simulink model "s_c_nbe_m32k"  (R2018a)
settings: Solver=VariableStepDiscrete  StartTime=0.0  StopTime=1000  RelTol=1e-3
undefined symbols (not defined in the file): fft_stages, n_taps, output_bits, pfb_coeff_gen_calc, xengbits
libraries: xbsIndex_r4 x23714, casper_library_misc x17, xps_library x4, casper_library_scopes x4, xbsReplacements_r4 x4
(part 8 of 171)

== system s_c_nbe_m32k/cd_hmc ==
  note: new delay values/enables come aligned
      | with data, need to be one cycle before
      | so new delay value gets loaded at the
      | same time as data, so delay data path
      | by one cycle
  sync_in : Inport
  din : Inport  Port=2
  en : Inport  Port=3
  delay_val : Inport  Port=4
  load_val : Inport  Port=5
  sync_in1 : Inport  Port=6
  din1 : Inport  Port=7
  en1 : Inport  Port=8
  delay_val1 : Inport  Port=9
  load_val1 : Inport  Port=10
  Constant : xbsIndex_r4/Constant  const=2^(n_bits_fft-3-1)  gui_display_data_type=Fixed-point  arith_type=Unsigned  n_bits=n_bits_fft-3  bin_pt=0  preci_type=Single  exp_width=8  frac_width=24  explicit_period=on  period=1  equ=P=C  opselect=C  inp2=PCIN>>17  opr=+  inp1=P  carry=CIN  dbl_ovrd=off  block_type=constant
  Constant1 : xbsIndex_r4/Constant  const=2^(n_bits_fft-3-1)  gui_display_data_type=Fixed-point  arith_type=Unsigned  n_bits=n_bits_fft-3  bin_pt=0  preci_type=Single  exp_width=8  frac_width=24  explicit_period=on  period=1  equ=P=C  opselect=C  inp2=PCIN>>17  opr=+  inp1=P  carry=CIN  dbl_ovrd=off  block_type=constant
  Constant2 : xbsIndex_r4/Constant  const=0  gui_display_data_type=Boolean  arith_type=Boolean  n_bits=1  bin_pt=0  preci_type=Single  exp_width=8  frac_width=24  explicit_period=on  period=1  equ=P=C  opselect=C  inp2=PCIN>>17  opr=+  inp1=P  carry=CIN  dbl_ovrd=off  block_type=constant
      settings: block_version=11.4
  Constant53 : xbsIndex_r4/Constant  const=0  gui_display_data_type=Boolean  arith_type=Boolean  n_bits=1  bin_pt=0  preci_type=Single  exp_width=8  frac_width=24  explicit_period=on  period=1  equ=P=C  opselect=C  inp2=PCIN>>17  opr=+  inp1=P  carry=CIN  dbl_ovrd=off  block_type=constant
      settings: block_version=11.4
  Delay : xbsIndex_r4/Delay  rst=off  infoeditControl=Selection of Reset will increase slice count due to use of real FFs and instead of SRLs  en=on  latency=1  reg_retiming=off  dbl_ovrd=off  block_type=delay
  Delay{1..4,6..19,21..34,36..39} (36 alike) : xbsIndex_r4/Delay  rst=off  infoeditControl=Selection of Reset will increase slice count due to use of real FFs and instead of SRLs  en=off  latency=1  reg_retiming=on  dbl_ovrd=off  block_type=delay
  Delay20 : xbsIndex_r4/Delay  rst=off  infoeditControl=Selection of Reset will increase slice count due to use of real FFs and instead of SRLs  en=on  latency=1  reg_retiming=off  dbl_ovrd=off  block_type=delay
  Delay35 : xbsIndex_r4/Delay  rst=off  infoeditControl=Selection of Reset will increase slice count due to use of real FFs and instead of SRLs  en=off  latency=1  reg_retiming=off  dbl_ovrd=off  block_type=delay
  Delay5 : xbsIndex_r4/Delay  rst=off  infoeditControl=Selection of Reset will increase slice count due to use of real FFs and instead of SRLs  en=off  latency=1  reg_retiming=off  dbl_ovrd=off  block_type=delay
  Logical : xbsIndex_r4/Logical  logical_function=AND  inputs=2  en=off  latency=1  precision=Full  arith_type=Unsigned  n_bits=16  bin_pt=0  align_bp=on  dbl_ovrd=off  block_type=logical
  Logical1 : xbsIndex_r4/Logical  logical_function=AND  inputs=2  en=off  latency=1  precision=Full  arith_type=Unsigned  n_bits=16  bin_pt=0  align_bp=on  dbl_ovrd=off  block_type=logical
  Slice1 : xbsIndex_r4/Slice  nbits=4  boolean_output=off  mode=Two Bit Locations  bit1=0  base1=MSB of Input  bit0=4  base0=LSB of Input  dbl_ovrd=off  block_type=slice
  Slice2 : xbsIndex_r4/Slice  nbits=4  boolean_output=off  mode=Two Bit Locations  bit1=0  base1=MSB of Input  bit0=4  base0=LSB of Input  dbl_ovrd=off  block_type=slice
  bus_expand1 : Subsystem  mask(bus_expand){mode=divisions of arbitrary size, outputNum=1, outputWidth=[64 64 16 16], outputBinaryPt=[32 32 15 15], outputArithmeticType=[1 1 1 1], show_format=off, outputToWorkspace=off, variablePrefix=out, outputToModelAsWell=on}
      mask prompts: outputNum "Number of outputs:"; outputWidth "Output width [msb ... lsb]:"; outputBinaryPt "Output binary point position [msb ... lsb]:"; outputArithmeticType "Output arithmetic type (ufix=0, fix=1, bool=2) [msb ... lsb]:"; show_format "Print format string?"; outputToWorkspace "Output to workspace?"; variablePrefix "Variable name prefix:"; outputToModelAsWell "Output to model as well?"
      mask help:
      | Expands a 'bus' made using a bus_create or Xilinx
      | concat block.
      | The input will be divided into the specified number
      | of outputs with the specified arithmetic types.
      | Divisions are made from most significant bit.
      mask init: same as s_c_nbe_m32k/bus_expand1
      settings: AttributesFormatString=4 outputs
      mask TypeOptions mode: divisions of equal size | divisions of arbitrary size
      mask Callback mode: bus_expand_callback();
      mask Callback outputWidth: bus_expand_callback();
      mask Callback outputToWorkspace: bus_expand_callback();
  bus_expand2 : Subsystem  mask(bus_expand){mode=divisions of arbitrary size, outputNum=1, outputWidth=[64 64 16 16], outputBinaryPt=[32 32 15 15], outputArithmeticType=[1 1 1 1], show_format=off, outputToWorkspace=off, variablePrefix=out, outputToModelAsWell=on}
      mask prompts: outputNum "Number of outputs:"; outputWidth "Output width [msb ... lsb]:"; outputBinaryPt "Output binary point position [msb ... lsb]:"; outputArithmeticType "Output arithmetic type (ufix=0, fix=1, bool=2) [msb ... lsb]:"; show_format "Print format string?"; outputToWorkspace "Output to workspace?"; variablePrefix "Variable name prefix:"; outputToModelAsWell "Output to model as well?"
      mask help:
      | Expands a 'bus' made using a bus_create or Xilinx
      | concat block.
      | The input will be divided into the specified number
      | of outputs with the specified arithmetic types.
      | Divisions are made from most significant bit.
      mask init: same as s_c_nbe_m32k/bus_expand1
      settings: AttributesFormatString=4 outputs
      mask TypeOptions mode: divisions of equal size | divisions of arbitrary size
      mask Callback mode: bus_expand_callback();
      mask Callback outputWidth: bus_expand_callback();
      mask Callback outputToWorkspace: bus_expand_callback();
  delay_gen0 : Subsystem  mask{fft_len=n_bits_fft-1, add_latency=1, data_bits=10 * 8, n_bits_index=n_bits_fft-3, lookup_bits=11, cd_bits=n_bits_cd, delay_bits=n_bits_cd+32, delay_bin_pt=32, max_delay_rate=23, min_delay_rate=38, phase_bits=16, max_phase_rate=23, min_phase_rate=38}
      mask prompts: fft_len "Effective FFT size (2^?)"; add_latency "Add latency"; data_bits "Data width"; n_bits_index "Index width"; lookup_bits "DDS lookup table resolution (2*pi/2^?)"; cd_bits "Coarse delay range (2^? bits)"; delay_bits "Input delay resolution (bits)"; delay_bin_pt "Input delay binary point"; max_delay_rate "Max delay update rate (1/2^? samples/sample)"; min_delay_rate "Min (non-zero) delay update rate (1/2^? samples/sample)"; phase_bits "Input phase resolution (2*pi/2^? radians)"; max_phase_rate "Max phase update rate (1/2^? radians/sample)"; min_phase_rate "Min (non-zero) phase rate (1/2^? radians/sample)"
  delay_gen1 : Subsystem  mask{fft_len=n_bits_fft-1, add_latency=1, data_bits=10 * 8, n_bits_index=n_bits_fft-3, lookup_bits=11, cd_bits=n_bits_cd, delay_bits=n_bits_cd+15, delay_bin_pt=15, max_delay_rate=23, min_delay_rate=38, phase_bits=16, max_phase_rate=23, min_phase_rate=38}
      mask prompts: fft_len "Effective FFT size (2^?)"; add_latency "Add latency"; data_bits "Data width"; n_bits_index "Index width"; lookup_bits "DDS lookup table resolution (2*pi/2^?)"; cd_bits "Coarse delay range (2^? bits)"; delay_bits "Input delay resolution (bits)"; delay_bin_pt "Input delay binary point"; max_delay_rate "Max delay update rate (1/2^? samples/sample)"; min_delay_rate "Min (non-zero) delay update rate (1/2^? samples/sample)"; phase_bits "Input phase resolution (2*pi/2^? radians)"; max_phase_rate "Max phase update rate (1/2^? radians/sample)"; min_phase_rate "Min (non-zero) phase rate (1/2^? radians/sample)"
  edge_detect : Subsystem  mask(edge_detect){edge=Rising, polarity=Active High, x_in=[0 0.08 0.08 0.16 0.16 0.24 0.24 0.32 0.32 0.4], y_in=[-1 -1  1  1  1  1  1  1  1  1], x_out=[0.6 0.68 0.68 0.76 0.76 0.84 0.84 0.92 0.92 1], y_out=[-1 -1  1  1 -1 -1 -1 -1 -1 -1]}
      mask prompts: edge "Edge Type"; polarity "Output Polarity"; x_in "Input X Positions"; y_in "Input Y Positions"; x_out "Output X Positions"; y_out "Output Y Positions"
      mask help: Output is active for one-cycle after each edge of the specified type (i.e. rising, falling or both).
      mask init: same as s_c_nbe_m32k/edge_detect1
      settings: AttributesFormatString=|
      | rising edges
      | active high
      mask Help: Output is active for one-cycle after each edge of the specified type (i.e. rising, falling, or both).  Latency is zero.
      mask TypeOptions edge: Rising | Falling | Both
      mask TypeOptions polarity: Active High | Active Low
      mask Display:
      | plot(x_in_num,0.5+y_in_num*0.2);
      | plot(x_out_num,0.5+y_out_num*0.2);
  edge_detect1 : Subsystem  mask(edge_detect){edge=Rising, polarity=Active High, x_in=[0 0.08 0.08 0.16 0.16 0.24 0.24 0.32 0.32 0.4], y_in=[-1 -1  1  1  1  1  1  1  1  1], x_out=[0.6 0.68 0.68 0.76 0.76 0.84 0.84 0.92 0.92 1], y_out=[-1 -1  1  1 -1 -1 -1 -1 -1 -1]}
      mask prompts: edge "Edge Type"; polarity "Output Polarity"; x_in "Input X Positions"; y_in "Input Y Positions"; x_out "Output X Positions"; y_out "Output Y Positions"
      mask help: Output is active for one-cycle after each edge of the specified type (i.e. rising, falling or both).
      mask init: same as s_c_nbe_m32k/edge_detect1
      settings: AttributesFormatString=|
      | rising edges
      | active high
      mask Help: Output is active for one-cycle after each edge of the specified type (i.e. rising, falling, or both).  Latency is zero.
      mask TypeOptions edge: Rising | Falling | Both
      mask TypeOptions polarity: Active High | Active Low
      mask Display:
      | plot(x_in_num,0.5+y_in_num*0.2);
      | plot(x_out_num,0.5+y_out_num*0.2);
  fft_index : xbsIndex_r4/Counter  cnt_type=Free Running  cnt_to=Inf  operation=Up  start_count=2^(n_bits_fft-4)  cnt_by_val=1  arith_type=Unsigned  n_bits=n_bits_fft-3  bin_pt=0  load_pin=off  rst=on  en=on  explicit_period=on  period=1  use_behavioral_HDL=on  implementation=Fabric  dbl_ovrd=off  block_type=counter
  fft_index1 : xbsIndex_r4/Counter  cnt_type=Free Running  cnt_to=Inf  operation=Up  start_count=2^(n_bits_fft-4)  cnt_by_val=1  arith_type=Unsigned  n_bits=n_bits_fft-3  bin_pt=0  load_pin=off  rst=on  en=on  explicit_period=on  period=1  use_behavioral_HDL=on  implementation=Fabric  dbl_ovrd=off  block_type=counter
  first : xbsIndex_r4/Relational  mode=a=b  op_type=Bool  en=off  latency=1  dbl_ovrd=off  block_type=relational
  first1 : xbsIndex_r4/Relational  mode=a=b  op_type=Bool  en=off  latency=1  dbl_ovrd=off  block_type=relational
  hmc_delay : Subsystem  mask{n_bits_max_delay=n_bits_cd-4}
      mask prompts: n_bits_max_delay "Maximum delay (2^?)"
      mask help:
      | Writes vectors in as rows in matrix and reads
      | out columns. Order in which columns read out
      | determined by 'Output column order' parameter.
      mask init:
      | % set_param([gcb, '/qdr'], 'which_qdr', which_qdr);
  req_hmc_cd0 : Subsystem  Tag=xps:sw_reg  AncestorBlock=xps_library/Memory/software_register  mask(swreg){io_dir=To Processor, io_delay=0, init_val=0, sample_period=1, names=reg, bitwidths=28, bin_pts=0, arith_types=0, sim_port=off, show_format=on}
      mask prompts: io_dir "I/O direction"; io_delay "I/O delay"; init_val "Initial Value"; sample_period "Sample period"; names "Bitfield names [msb...lsb]"; bitwidths "Bitfield widths"; bin_pts "Bitfield binary pts"; arith_types "Bitfield types, ufix=0, fix=1, bool=2"; sim_port "Provide sim input/output?"; show_format "Print format string?"
      mask help: A 32-bit software-accessible register. Can be divided into bitfields of varying widths and types using the fields in the block mask.
      mask init:
      | swreg_init(gcb)
      settings: AttributesFormatString=1output:uf28.0 = 28 bits
      mask TypeOptions io_dir: To Processor | From Processor
      mask Callback io_dir:
      | mask_enables = get_param(gcb, 'MaskEnables');
      | mask_names = get_param(gcb, 'MaskNames');
      | if strcmp(get_param(gcb, 'io_dir'), 'To Processor'),
      |     mask_enables{ismember(mask_names, 'sample_period')} = 'off';
      | else
      |     mask_enables{ismember(mask_names, 'sample_period')} = 'on';
      | end
      | set_param(gcb, 'MaskEnables', mask_enables);
      mask DialogControl ParameterTabVar0 Prompt: Setup
  req_hmc_cd1 : Subsystem  Tag=xps:sw_reg  AncestorBlock=xps_library/Memory/software_register  mask(swreg){io_dir=To Processor, io_delay=0, init_val=0, sample_period=1, names=reg, bitwidths=28, bin_pts=0, arith_types=0, sim_port=off, show_format=on}
      mask prompts: io_dir "I/O direction"; io_delay "I/O delay"; init_val "Initial Value"; sample_period "Sample period"; names "Bitfield names [msb...lsb]"; bitwidths "Bitfield widths"; bin_pts "Bitfield binary pts"; arith_types "Bitfield types, ufix=0, fix=1, bool=2"; sim_port "Provide sim input/output?"; show_format "Print format string?"
      mask help: A 32-bit software-accessible register. Can be divided into bitfields of varying widths and types using the fields in the block mask.
      mask init:
      | swreg_init(gcb)
      settings: AttributesFormatString=1output:uf28.0 = 28 bits
      mask TypeOptions io_dir: To Processor | From Processor
      mask Callback io_dir:
      | mask_enables = get_param(gcb, 'MaskEnables');
      | mask_names = get_param(gcb, 'MaskNames');
      | if strcmp(get_param(gcb, 'io_dir'), 'To Processor'),
      |     mask_enables{ismember(mask_names, 'sample_period')} = 'off';
      | else
      |     mask_enables{ismember(mask_names, 'sample_period')} = 'on';
      | end
      | set_param(gcb, 'MaskEnables', mask_enables);
      mask DialogControl ParameterTabVar0 Prompt: Setup
  sync_out : Outport
  dout0 : Outport  Port=2
  dout1 : Outport  Port=3
  dvalid : Outport  Port=4
  hmc_error : Outport  Port=5
  wires:
  Slice1/1 -> Delay/1
  hmc_delay/1(sync_out) -> [sync_out]  "dw_sync"
  hmc_delay/2(data_out0) -> [data0]
  hmc_delay/3(dv) -> [dvalid]  "dw_en"
  hmc_delay/4(error) -> [hmc_error]
  [hmc_error] -> hmc_error/1
  [sync_out] -> sync_out/1
  [data0] -> dout0/1
  [dvalid] -> dvalid/1
  Delay/1 -> hmc_delay/4(delay_pol0), req_hmc_cd0/1(out_reg)  "delay_in"
  Delay5/1 -> hmc_delay/1(sync)
  din/1 -> Delay2/1
  sync_in/1 -> Delay1/1, fft_index/1
  Constant53/1 -> delay_gen0/11(invert_slope)
  fft_index/1 -> Delay3/1, first/2
  delay_gen0/1(sync_out) -> Delay5/1
  en/1 -> Delay4/1, fft_index/2
  delay_gen0/2(dout) -> hmc_delay/2(data_in_pol0)
  Constant/1 -> first/1
  first/1 -> Logical/1
  Delay1/1 -> Delay19/1
  Delay3/1 -> Delay11/1
  Delay4/1 -> Logical/2, Delay12/1
  load_val/1 -> Delay6/1
  delay_gen0/4(dvalid) -> hmc_delay/3(en_in)
  Delay6/1 -> Delay13/1
  Delay7/1 -> Delay14/1
  Delay8/1 -> Delay15/1
  Delay9/1 -> Delay16/1
  Delay18/1 -> Delay17/1
  Delay2/1 -> Delay10/1
  Delay19/1 -> delay_gen0/1(sync_in)
  Delay10/1 -> delay_gen0/3(din)
  Delay11/1 -> delay_gen0/4(idx_in)
  Delay12/1 -> delay_gen0/5(den)
  Delay13/1 -> delay_gen0/6(load)
  Delay14/1 -> delay_gen0/7(phase)
  Delay15/1 -> delay_gen0/8(d/dt_phase)
  Delay16/1 -> delay_gen0/9(delay)
  Delay17/1 -> delay_gen0/10(d/dt_delay)
  Logical/1 -> edge_detect/1(in)
  edge_detect/1(out) -> delay_gen0/2(init)
  bus_expand1/1(msb_out4) -> Delay9/1
  bus_expand1/2(out3) -> Delay18/1
  bus_expand1/3(out2) -> Delay7/1
  bus_expand1/4(lsb_out1) -> Delay8/1
  delay_val/1 -> bus_expand1/1(bus_in)
  delay_gen0/5(cd_o) -> Slice1/1
  delay_gen0/8(load_out) -> Delay/2
  [data1] -> dout1/1
  hmc_delay/5(data_out1) -> [data1]
  Slice2/1 -> Delay20/1
  Delay20/1 -> hmc_delay/8(delay_pol1), req_hmc_cd1/1(out_reg)  "delay_in"
  din1/1 -> Delay32/1
  sync_in1/1 -> fft_index1/1, Delay21/1
  Constant2/1 -> delay_gen1/11(invert_slope)
  fft_index1/1 -> first1/2, Delay33/1
  delay_gen1/1(sync_out) -> Delay35/1
  en1/1 -> fft_index1/2, Delay34/1
  Constant1/1 -> first1/1
  first1/1 -> Logical1/1
  Delay21/1 -> Delay31/1
  Delay33/1 -> Delay23/1
  Delay34/1 -> Delay24/1, Logical1/2
  load_val1/1 -> Delay36/1
  Delay36/1 -> Delay25/1
  Delay37/1 -> Delay26/1
  Delay38/1 -> Delay27/1
  Delay39/1 -> Delay28/1
  Delay30/1 -> Delay29/1
  Delay32/1 -> Delay22/1
  Delay31/1 -> delay_gen1/1(sync_in)
  Delay22/1 -> delay_gen1/3(din)
  Delay23/1 -> delay_gen1/4(idx_in)
  Delay24/1 -> delay_gen1/5(den)
  Delay25/1 -> delay_gen1/6(load)
  Delay26/1 -> delay_gen1/7(phase)
  Delay27/1 -> delay_gen1/8(d/dt_phase)
  Delay28/1 -> delay_gen1/9(delay)
  Delay29/1 -> delay_gen1/10(d/dt_delay)
  Logical1/1 -> edge_detect1/1(in)
  edge_detect1/1(out) -> delay_gen1/2(init)
  bus_expand2/1(msb_out4) -> Delay39/1
  bus_expand2/2(out3) -> Delay30/1
  bus_expand2/3(out2) -> Delay37/1
  bus_expand2/4(lsb_out1) -> Delay38/1
  delay_val1/1 -> bus_expand2/1(bus_in)
  delay_gen1/5(cd_o) -> Slice2/1
  delay_gen1/8(load_out) -> Delay20/2
  Delay35/1 -> hmc_delay/5(sync1)
  delay_gen1/4(dvalid) -> hmc_delay/7(en)
  delay_gen1/2(dout) -> hmc_delay/6(data_in_pol1)

== system s_c_nbe_m32k/cd_in_dv_rate ==
  out_reg : Inport
  assert_reg : xbsIndex_r4/Assert  assert_type=on  type_source=Explicitly  gui_display_data_type=Fixed-point  arith_type=Unsigned  n_bits=32  bin_pt=0  preci_type=Single  exp_width=8  frac_width=24  assert_rate=off  rate_source=Explicitly  period=1  output_port=on  block_type=assert
  cast_gw : xbsIndex_r4/Convert  gui_display_data_type=Fixed-point  arith_type=Unsigned  n_bits=32  bin_pt=0  float_type=Single  exp_bits=8  fraction_bits=24  quantization=Truncate  overflow=Wrap  en=off  latency=1  pipeline=off  dbl_ovrd=off  block_type=convert
  io_delay : xbsIndex_r4/Delay  rst=off  infoeditControl=Selection of Reset will increase slice count due to use of real FFs and instead of SRLs  en=off  latency=0  reg_retiming=on  dbl_ovrd=off  block_type=delay
  reint1 : xbsIndex_r4/Reinterpret  force_arith_type=on  arith_type=Unsigned  force_bin_pt=on  bin_pt=0  block_type=reinterpret
  s_c_nbe_m32k_v9_cd_in_dv_rate_user_data_in : xbsIndex_r4/Gateway Out  inherit_from_input=off  hdl_port=on  rows=1  columns=1  UseAsDAC=off  DACChannel='1'  interface=None  automatic_assignment=on  address_offset=hex2dec('00')  intf_name=''  intf_description=''  timing_constraint=None  locs_specified=off  LOCs={}  io_standard={}  block_type=gatewayout
  sim_out : Terminator
  wires:
  io_delay/1 -> cast_gw/1
  cast_gw/1 -> s_c_nbe_m32k_v9_cd_in_dv_rate_user_data_in/1
  s_c_nbe_m32k_v9_cd_in_dv_rate_user_data_in/1 -> sim_out/1
  out_reg/1 -> assert_reg/1
  assert_reg/1 -> reint1/1
  reint1/1 -> io_delay/1

== system s_c_nbe_m32k/cd_out_dv_rate ==
  out_reg : Inport
  assert_reg : xbsIndex_r4/Assert  assert_type=on  type_source=Explicitly  gui_display_data_type=Fixed-point  arith_type=Unsigned  n_bits=32  bin_pt=0  preci_type=Single  exp_width=8  frac_width=24  assert_rate=off  rate_source=Explicitly  period=1  output_port=on  block_type=assert
  cast_gw : xbsIndex_r4/Convert  gui_display_data_type=Fixed-point  arith_type=Unsigned  n_bits=32  bin_pt=0  float_type=Single  exp_bits=8  fraction_bits=24  quantization=Truncate  overflow=Wrap  en=off  latency=1  pipeline=off  dbl_ovrd=off  block_type=convert
  io_delay : xbsIndex_r4/Delay  rst=off  infoeditControl=Selection of Reset will increase slice count due to use of real FFs and instead of SRLs  en=off  latency=0  reg_retiming=on  dbl_ovrd=off  block_type=delay
  reint1 : xbsIndex_r4/Reinterpret  force_arith_type=on  arith_type=Unsigned  force_bin_pt=on  bin_pt=0  block_type=reinterpret
  s_c_nbe_m32k_v9_cd_out_dv_rate_user_data_in : xbsIndex_r4/Gateway Out  inherit_from_input=off  hdl_port=on  rows=1  columns=1  UseAsDAC=off  DACChannel='1'  interface=None  automatic_assignment=on  address_offset=hex2dec('00')  intf_name=''  intf_description=''  timing_constraint=None  locs_specified=off  LOCs={}  io_standard={}  block_type=gatewayout
  sim_out : Terminator
  wires:
  io_delay/1 -> cast_gw/1
  cast_gw/1 -> s_c_nbe_m32k_v9_cd_out_dv_rate_user_data_in/1
  s_c_nbe_m32k_v9_cd_out_dv_rate_user_data_in/1 -> sim_out/1
  out_reg/1 -> assert_reg/1
  assert_reg/1 -> reint1/1
  reint1/1 -> io_delay/1

== system s_c_nbe_m32k/cd_status ==
  out_sync80 : Inport
  out_sync80_1 : Inport  Port=2
  out_hmc_sync_out : Inport  Port=3
  assert_hmc_sync_out : xbsIndex_r4/Assert  assert_type=on  type_source=Explicitly  gui_display_data_type=Fixed-point  arith_type=Unsigned  n_bits=8  bin_pt=0  preci_type=Single  exp_width=8  frac_width=24  assert_rate=off  rate_source=Explicitly  period=1  output_port=on  block_type=assert
  assert_sync80 : xbsIndex_r4/Assert  assert_type=on  type_source=Explicitly  gui_display_data_type=Fixed-point  arith_type=Unsigned  n_bits=8  bin_pt=0  preci_type=Single  exp_width=8  frac_width=24  assert_rate=off  rate_source=Explicitly  period=1  output_port=on  block_type=assert
  assert_sync80_1 : xbsIndex_r4/Assert  assert_type=on  type_source=Explicitly  gui_display_data_type=Fixed-point  arith_type=Unsigned  n_bits=8  bin_pt=0  preci_type=Single  exp_width=8  frac_width=24  assert_rate=off  rate_source=Explicitly  period=1  output_port=on  block_type=assert
  cast_gw : xbsIndex_r4/Convert  gui_display_data_type=Fixed-point  arith_type=Unsigned  n_bits=32  bin_pt=0  float_type=Single  exp_bits=8  fraction_bits=24  quantization=Truncate  overflow=Wrap  en=off  latency=1  pipeline=off  dbl_ovrd=off  block_type=convert
  concatenate : xbsIndex_r4/Concat  num_inputs=3  dbl_ovrd=off  block_type=concat
  io_delay : xbsIndex_r4/Delay  rst=off  infoeditControl=Selection of Reset will increase slice count due to use of real FFs and instead of SRLs  en=off  latency=0  reg_retiming=on  dbl_ovrd=off  block_type=delay
  reint1 : xbsIndex_r4/Reinterpret  force_arith_type=on  arith_type=Unsigned  force_bin_pt=on  bin_pt=0  block_type=reinterpret
  reint2 : xbsIndex_r4/Reinterpret  force_arith_type=on  arith_type=Unsigned  force_bin_pt=on  bin_pt=0  block_type=reinterpret
  reint3 : xbsIndex_r4/Reinterpret  force_arith_type=on  arith_type=Unsigned  force_bin_pt=on  bin_pt=0  block_type=reinterpret
  s_c_nbe_m32k_v9_cd_status_user_data_in : xbsIndex_r4/Gateway Out  inherit_from_input=off  hdl_port=on  rows=1  columns=1  UseAsDAC=off  DACChannel='1'  interface=None  automatic_assignment=on  address_offset=hex2dec('00')  intf_name=''  intf_description=''  timing_constraint=None  locs_specified=off  LOCs={}  io_standard={}  block_type=gatewayout
  sim_out : Terminator
  wires:
  concatenate/1 -> io_delay/1
  io_delay/1 -> cast_gw/1
  cast_gw/1 -> s_c_nbe_m32k_v9_cd_status_user_data_in/1
  s_c_nbe_m32k_v9_cd_status_user_data_in/1 -> sim_out/1
  out_sync80/1 -> assert_sync80/1
  assert_sync80/1 -> reint1/1
  reint1/1 -> concatenate/1
  out_sync80_1/1 -> assert_sync80_1/1
  assert_sync80_1/1 -> reint2/1
  reint2/1 -> concatenate/2
  out_hmc_sync_out/1 -> assert_hmc_sync_out/1
  assert_hmc_sync_out/1 -> reint3/1
  reint3/1 -> concatenate/3

== system s_c_nbe_m32k/complexify ==
  In1 : Inport
  Constant : xbsIndex_r4/Constant  const=0  gui_display_data_type=Fixed-point  arith_type=Signed (2's comp)  n_bits=10  bin_pt=9  preci_type=Single  exp_width=8  frac_width=24  explicit_period=on  period=1  equ=P=C  opselect=C  inp2=PCIN>>17  opr=+  inp1=P  carry=CIN  dbl_ovrd=off  block_type=constant
  bus_create : Subsystem  mask(bus_create){inputNum=8}
      mask prompts: inputNum "Number of inputs:"
      mask init:
      | bus_create_init(gcb,...
      |     'inputNum', inputNum);
  bus_expand6 : Subsystem  mask(bus_expand){mode=divisions of equal size, outputNum=8, outputWidth=10, outputBinaryPt=9, outputArithmeticType=1, show_format=off, outputToWorkspace=off, variablePrefix=out, outputToModelAsWell=on}
      mask prompts: outputNum "Number of outputs:"; outputWidth "Output width:"; outputBinaryPt "Output binary point position:"; outputArithmeticType "Output arithmetic type (ufix=0, fix=1, bool=2):"; show_format "Print format string?"; outputToWorkspace "Output to workspace?"; variablePrefix "Variable name prefix:"; outputToModelAsWell "Output to model as well?"
      mask help:
      | Expands a 'bus' made using a bus_create or Xilinx
      | concat block.
      | The input will be divided into the specified number
      | of outputs with the specified arithmetic types.
      | Divisions are made from most significant bit.
      mask init: same as s_c_nbe_m32k/bus_expand1
      settings: AttributesFormatString=8 outputs
      mask TypeOptions mode: divisions of equal size | divisions of arbitrary size
      mask Callback mode: bus_expand_callback();
      mask Callback outputWidth: bus_expand_callback();
      mask Callback outputToWorkspace: bus_expand_callback();
  ri_to_c : Subsystem  mask(ri_to_c){}
      mask help:
      | Concatenates real and imaginary inputs into a complex output.
      | Useful for simplifying interconnects.
      | See also: Complex to Real-Imag (c_to_ri)
      mask Help: eval('xlWeb(''http://casper.berkeley.edu/wiki/Ri_to_c'')')
  ri_to_c1 : Subsystem  mask(ri_to_c){}
      mask help:
      | Concatenates real and imaginary inputs into a complex output.
      | Useful for simplifying interconnects.
      | See also: Complex to Real-Imag (c_to_ri)
      mask Help: eval('xlWeb(''http://casper.berkeley.edu/wiki/Ri_to_c'')')
  ri_to_c2 : Subsystem  mask(ri_to_c){}
      mask help:
      | Concatenates real and imaginary inputs into a complex output.
      | Useful for simplifying interconnects.
      | See also: Complex to Real-Imag (c_to_ri)
      mask Help: eval('xlWeb(''http://casper.berkeley.edu/wiki/Ri_to_c'')')
  ri_to_c3 : Subsystem  mask(ri_to_c){}
      mask help:
      | Concatenates real and imaginary inputs into a complex output.
      | Useful for simplifying interconnects.
      | See also: Complex to Real-Imag (c_to_ri)
      mask Help: eval('xlWeb(''http://casper.berkeley.edu/wiki/Ri_to_c'')')
  ri_to_c4 : Subsystem  mask(ri_to_c){}
      mask help:
      | Concatenates real and imaginary inputs into a complex output.
      | Useful for simplifying interconnects.
      | See also: Complex to Real-Imag (c_to_ri)
      mask Help: eval('xlWeb(''http://casper.berkeley.edu/wiki/Ri_to_c'')')
  ri_to_c5 : Subsystem  mask(ri_to_c){}
      mask help:
      | Concatenates real and imaginary inputs into a complex output.
      | Useful for simplifying interconnects.
      | See also: Complex to Real-Imag (c_to_ri)
      mask Help: eval('xlWeb(''http://casper.berkeley.edu/wiki/Ri_to_c'')')
  ri_to_c6 : Subsystem  mask(ri_to_c){}
      mask help:
      | Concatenates real and imaginary inputs into a complex output.
      | Useful for simplifying interconnects.
      | See also: Complex to Real-Imag (c_to_ri)
      mask Help: eval('xlWeb(''http://casper.berkeley.edu/wiki/Ri_to_c'')')
  ri_to_c7 : Subsystem  mask(ri_to_c){}
      mask help:
      | Concatenates real and imaginary inputs into a complex output.
      | Useful for simplifying interconnects.
      | See also: Complex to Real-Imag (c_to_ri)
      mask Help: eval('xlWeb(''http://casper.berkeley.edu/wiki/Ri_to_c'')')
  Out1 : Outport
  wires:
  bus_expand6/6(out3) -> ri_to_c5/1(re)
  bus_expand6/4(out5) -> ri_to_c3/1(re)
  Constant/1 -> ri_to_c1/2(im), ri_to_c2/2(im), ri_to_c3/2(im), ri_to_c4/2(im), ri_to_c5/2(im), ri_to_c6/2(im), ri_to_c7/2(im), ri_to_c/2(im)
  ri_to_c5/1(c) -> bus_create/6(in6)
  ri_to_c2/1(c) -> bus_create/3(in3)
  In1/1 -> bus_expand6/1(bus_in)
  ri_to_c1/1(c) -> bus_create/2(in2)
  bus_expand6/3(out6) -> ri_to_c2/1(re)
  bus_expand6/1(msb_out8) -> ri_to_c/1(re)
  bus_expand6/5(out4) -> ri_to_c4/1(re)
  ri_to_c6/1(c) -> bus_create/7(in7)
  bus_expand6/8(lsb_out1) -> ri_to_c7/1(re)
  bus_create/1(bus_out) -> Out1/1
  bus_expand6/2(out7) -> ri_to_c1/1(re)
  ri_to_c3/1(c) -> bus_create/4(in4)
  ri_to_c4/1(c) -> bus_create/5(in5)
  ri_to_c/1(c) -> bus_create/1(in1)
  ri_to_c7/1(c) -> bus_create/8(in8)
  bus_expand6/7(out2) -> ri_to_c6/1(re)

== system s_c_nbe_m32k/complexify1 ==
  In1 : Inport
  Constant : xbsIndex_r4/Constant  const=0  gui_display_data_type=Fixed-point  arith_type=Signed (2's comp)  n_bits=10  bin_pt=9  preci_type=Single  exp_width=8  frac_width=24  explicit_period=on  period=1  equ=P=C  opselect=C  inp2=PCIN>>17  opr=+  inp1=P  carry=CIN  dbl_ovrd=off  block_type=constant
  bus_create : Subsystem  mask(bus_create){inputNum=8}
      mask prompts: inputNum "Number of inputs:"
      mask init:
      | bus_create_init(gcb,...
      |     'inputNum', inputNum);
  bus_expand6 : Subsystem  mask(bus_expand){mode=divisions of equal size, outputNum=8, outputWidth=10, outputBinaryPt=9, outputArithmeticType=1, show_format=off, outputToWorkspace=off, variablePrefix=out, outputToModelAsWell=on}
      mask prompts: outputNum "Number of outputs:"; outputWidth "Output width:"; outputBinaryPt "Output binary point position:"; outputArithmeticType "Output arithmetic type (ufix=0, fix=1, bool=2):"; show_format "Print format string?"; outputToWorkspace "Output to workspace?"; variablePrefix "Variable name prefix:"; outputToModelAsWell "Output to model as well?"
      mask help:
      | Expands a 'bus' made using a bus_create or Xilinx
      | concat block.
      | The input will be divided into the specified number
      | of outputs with the specified arithmetic types.
      | Divisions are made from most significant bit.
      mask init: same as s_c_nbe_m32k/bus_expand1
      settings: AttributesFormatString=8 outputs
      mask TypeOptions mode: divisions of equal size | divisions of arbitrary size
      mask Callback mode: bus_expand_callback();
      mask Callback outputWidth: bus_expand_callback();
      mask Callback outputToWorkspace: bus_expand_callback();
  ri_to_c : Subsystem  mask(ri_to_c){}
      mask help:
      | Concatenates real and imaginary inputs into a complex output.
      | Useful for simplifying interconnects.
      | See also: Complex to Real-Imag (c_to_ri)
      mask Help: eval('xlWeb(''http://casper.berkeley.edu/wiki/Ri_to_c'')')
  ri_to_c1 : Subsystem  mask(ri_to_c){}
      mask help:
      | Concatenates real and imaginary inputs into a complex output.
      | Useful for simplifying interconnects.
      | See also: Complex to Real-Imag (c_to_ri)
      mask Help: eval('xlWeb(''http://casper.berkeley.edu/wiki/Ri_to_c'')')
  ri_to_c2 : Subsystem  mask(ri_to_c){}
      mask help:
      | Concatenates real and imaginary inputs into a complex output.
      | Useful for simplifying interconnects.
      | See also: Complex to Real-Imag (c_to_ri)
      mask Help: eval('xlWeb(''http://casper.berkeley.edu/wiki/Ri_to_c'')')
  ri_to_c3 : Subsystem  mask(ri_to_c){}
      mask help:
      | Concatenates real and imaginary inputs into a complex output.
      | Useful for simplifying interconnects.
      | See also: Complex to Real-Imag (c_to_ri)
      mask Help: eval('xlWeb(''http://casper.berkeley.edu/wiki/Ri_to_c'')')
  ri_to_c4 : Subsystem  mask(ri_to_c){}
      mask help:
      | Concatenates real and imaginary inputs into a complex output.
      | Useful for simplifying interconnects.
      | See also: Complex to Real-Imag (c_to_ri)
      mask Help: eval('xlWeb(''http://casper.berkeley.edu/wiki/Ri_to_c'')')
  ri_to_c5 : Subsystem  mask(ri_to_c){}
      mask help:
      | Concatenates real and imaginary inputs into a complex output.
      | Useful for simplifying interconnects.
      | See also: Complex to Real-Imag (c_to_ri)
      mask Help: eval('xlWeb(''http://casper.berkeley.edu/wiki/Ri_to_c'')')
  ri_to_c6 : Subsystem  mask(ri_to_c){}
      mask help:
      | Concatenates real and imaginary inputs into a complex output.
      | Useful for simplifying interconnects.
      | See also: Complex to Real-Imag (c_to_ri)
      mask Help: eval('xlWeb(''http://casper.berkeley.edu/wiki/Ri_to_c'')')
  ri_to_c7 : Subsystem  mask(ri_to_c){}
      mask help:
      | Concatenates real and imaginary inputs into a complex output.
      | Useful for simplifying interconnects.
      | See also: Complex to Real-Imag (c_to_ri)
      mask Help: eval('xlWeb(''http://casper.berkeley.edu/wiki/Ri_to_c'')')
  Out1 : Outport
  wires:
  bus_expand6/7(out2) -> ri_to_c6/1(re)
  ri_to_c7/1(c) -> bus_create/8(in8)
  ri_to_c/1(c) -> bus_create/1(in1)
  ri_to_c4/1(c) -> bus_create/5(in5)
  ri_to_c3/1(c) -> bus_create/4(in4)
  bus_expand6/2(out7) -> ri_to_c1/1(re)
  bus_create/1(bus_out) -> Out1/1
  bus_expand6/8(lsb_out1) -> ri_to_c7/1(re)
  ri_to_c6/1(c) -> bus_create/7(in7)
  bus_expand6/5(out4) -> ri_to_c4/1(re)
  bus_expand6/1(msb_out8) -> ri_to_c/1(re)
  bus_expand6/3(out6) -> ri_to_c2/1(re)
  ri_to_c1/1(c) -> bus_create/2(in2)
  In1/1 -> bus_expand6/1(bus_in)
  ri_to_c2/1(c) -> bus_create/3(in3)
  ri_to_c5/1(c) -> bus_create/6(in6)
  Constant/1 -> ri_to_c/2(im), ri_to_c7/2(im), ri_to_c6/2(im), ri_to_c5/2(im), ri_to_c4/2(im), ri_to_c3/2(im), ri_to_c2/2(im), ri_to_c1/2(im)
  bus_expand6/4(out5) -> ri_to_c3/1(re)
  bus_expand6/6(out3) -> ri_to_c5/1(re)

== system s_c_nbe_m32k/control ==
  convert1_{1..13,15..17,19,21..24} (21 alike) : DataTypeConversion  OutDataTypeStr=fixdt('ufix1_En0')  LockScale=on
  convert1_14 : DataTypeConversion  OutDataTypeStr=fixdt('ufix3_En0')  LockScale=on
  convert1_18 : DataTypeConversion  OutDataTypeStr=fixdt('ufix2_En0')  LockScale=on
  convert1_20 : DataTypeConversion  OutDataTypeStr=fixdt('ufix2_En0')  LockScale=on
  convert2_{1..13,15..17,19,21..24} (21 alike) : DataTypeConversion  OutDataTypeStr=fixdt('ufix1_En0')  ConvertRealWorld=Stored Integer (SI)  LockScale=on
  convert2_14 : DataTypeConversion  OutDataTypeStr=fixdt('ufix3_En0')  ConvertRealWorld=Stored Integer (SI)  LockScale=on
  convert2_18 : DataTypeConversion  OutDataTypeStr=fixdt('ufix2_En0')  ConvertRealWorld=Stored Integer (SI)  LockScale=on
  convert2_20 : DataTypeConversion  OutDataTypeStr=fixdt('ufix2_En0')  ConvertRealWorld=Stored Integer (SI)  LockScale=on
  gain_1 : Gain  Gain=134217728
  gain_10 : Gain  Gain=262144
  gain_11 : Gain  Gain=131072
  gain_12 : Gain  Gain=65536
  gain_13 : Gain  Gain=32768
  gain_14 : Gain  Gain=4096
  gain_15 : Gain  Gain=2048
  gain_16 : Gain  Gain=1024
  gain_17 : Gain  Gain=512
  gain_18 : Gain  Gain=128
  gain_19 : Gain  Gain=64
  gain_2 : Gain  Gain=67108864
  gain_20 : Gain  Gain=16
  gain_21 : Gain  Gain=8
  gain_22 : Gain  Gain=4
  gain_23 : Gain  Gain=2
  gain_24 : Gain
  gain_3 : Gain  Gain=33554432
  gain_4 : Gain  Gain=16777216
  gain_5 : Gain  Gain=8388608
  gain_6 : Gain  Gain=4194304
  gain_7 : Gain  Gain=2097152
  gain_8 : Gain  Gain=1048576
  gain_9 : Gain  Gain=524288
  io_delay : xbsIndex_r4/Delay  rst=off  infoeditControl=Selection of Reset will increase slice count due to use of real FFs and instead of SRLs  en=off  latency=1  reg_retiming=on  dbl_ovrd=off  block_type=delay
  reint{10..11,13..15,18..20} (8 alike) : xbsIndex_r4/Reinterpret  force_arith_type=on  arith_type=Unsigned  force_bin_pt=on  bin_pt=0  block_type=reinterpret
  s_c_nbe_m32k_v9_control_user_data_out : xbsIndex_r4/Gateway In  gui_display_data_type=Fixed-point  arith_type=Unsigned  n_bits=32  bin_pt=0  preci_type=Single  exp_width=8  frac_width=24  rows=1  columns=1  quantization="Round  (unbiased: +/- Inf)"  overflow=Saturate  period=1  UseAsADC=off  ADCChannel='1'  interface=None  automatic_assignment=on  address_offset=hex2dec('00')  intf_name=''  intf_description=''  default_value=0  timing_constraint=None  locs_specified=off  LOCs={}  io_standard={}  inherit_from_input=off  hdl_port=on  dbl_ovrd=off  block_type=gatewayin
  sim_{1..24} (24 alike) : Constant  Value=0
  sim_add : Sum  Inputs=++++++++++++++++++++++++  OutDataTypeStr=uint32
  slice_adc_snap_arm : xbsIndex_r4/Slice  nbits=1  boolean_output=on  mode=Lower Bit Location + Width  bit1=0  base1=MSB of Input  bit0=19  base0=LSB of Input  dbl_ovrd=off  block_type=slice
  slice_adc_snap_trig_select : xbsIndex_r4/Slice  nbits=1  boolean_output=off  mode=Lower Bit Location + Width  bit1=0  base1=MSB of Input  bit0=18  base0=LSB of Input  dbl_ovrd=off  block_type=slice
  slice_auto_rst_enable : xbsIndex_r4/Slice  nbits=1  boolean_output=on  mode=Lower Bit Location + Width  bit1=0  base1=MSB of Input  bit0=1  base0=LSB of Input  dbl_ovrd=off  block_type=slice
  slice_cd_bypass : xbsIndex_r4/Slice  nbits=1  boolean_output=off  mode=Lower Bit Location + Width  bit1=0  base1=MSB of Input  bit0=15  base0=LSB of Input  dbl_ovrd=off  block_type=slice
  slice_cnt_rst : xbsIndex_r4/Slice  nbits=1  boolean_output=on  mode=Lower Bit Location + Width  bit1=0  base1=MSB of Input  bit0=21  base0=LSB of Input  dbl_ovrd=off  block_type=slice
  slice_ct_tvg_en : xbsIndex_r4/Slice  nbits=1  boolean_output=off  mode=Lower Bit Location + Width  bit1=0  base1=MSB of Input  bit0=17  base0=LSB of Input  dbl_ovrd=off  block_type=slice
  slice_force_gbe_txen : xbsIndex_r4/Slice  nbits=1  boolean_output=on  mode=Lower Bit Location + Width  bit1=0  base1=MSB of Input  bit0=9  base0=LSB of Input  dbl_ovrd=off  block_type=slice
  slice_gbe_cnt_rst : xbsIndex_r4/Slice  nbits=1  boolean_output=on  mode=Lower Bit Location + Width  bit1=0  base1=MSB of Input  bit0=20  base0=LSB of Input  dbl_ovrd=off  block_type=slice
  slice_gbe_rst : xbsIndex_r4/Slice  nbits=1  boolean_output=on  mode=Lower Bit Location + Width  bit1=0  base1=MSB of Input  bit0=25  base0=LSB of Input  dbl_ovrd=off  block_type=slice
  slice_gbe_stopmux : xbsIndex_r4/Slice  nbits=3  boolean_output=off  mode=Lower Bit Location + Width  bit1=0  base1=MSB of Input  bit0=12  base0=LSB of Input  dbl_ovrd=off  block_type=slice
  slice_gbe_txen : xbsIndex_r4/Slice  nbits=1  boolean_output=on  mode=Lower Bit Location + Width  bit1=0  base1=MSB of Input  bit0=24  base0=LSB of Input  dbl_ovrd=off  block_type=slice
  slice_local_time_capture : xbsIndex_r4/Slice  nbits=1  boolean_output=on  mode=Lower Bit Location + Width  bit1=0  base1=MSB of Input  bit0=3  base0=LSB of Input  dbl_ovrd=off  block_type=slice
  slice_local_time_source : xbsIndex_r4/Slice  nbits=2  boolean_output=off  mode=Lower Bit Location + Width  bit1=0  base1=MSB of Input  bit0=4  base0=LSB of Input  dbl_ovrd=off  block_type=slice
  slice_pfb_bypass : xbsIndex_r4/Slice  nbits=1  boolean_output=off  mode=Lower Bit Location + Width  bit1=0  base1=MSB of Input  bit0=11  base0=LSB of Input  dbl_ovrd=off  block_type=slice
  slice_pipeline_stall : xbsIndex_r4/Slice  nbits=1  boolean_output=on  mode=Lower Bit Location + Width  bit1=0  base1=MSB of Input  bit0=0  base0=LSB of Input  dbl_ovrd=off  block_type=slice
  slice_snap_reord_mux_we_sel : xbsIndex_r4/Slice  nbits=1  boolean_output=off  mode=Lower Bit Location + Width  bit1=0  base1=MSB of Input  bit0=6  base0=LSB of Input  dbl_ovrd=off  block_type=slice
  slice_snap_stop_mux_sel : xbsIndex_r4/Slice  nbits=2  boolean_output=off  mode=Lower Bit Location + Width  bit1=0  base1=MSB of Input  bit0=7  base0=LSB of Input  dbl_ovrd=off  block_type=slice
  slice_status_clr : xbsIndex_r4/Slice  nbits=1  boolean_output=on  mode=Lower Bit Location + Width  bit1=0  base1=MSB of Input  bit0=26  base0=LSB of Input  dbl_ovrd=off  block_type=slice
  slice_sys_rst : xbsIndex_r4/Slice  nbits=1  boolean_output=on  mode=Lower Bit Location + Width  bit1=0  base1=MSB of Input  bit0=27  base0=LSB of Input  dbl_ovrd=off  block_type=slice
  slice_time_diff_check_en : xbsIndex_r4/Slice  nbits=1  boolean_output=on  mode=Lower Bit Location + Width  bit1=0  base1=MSB of Input  bit0=2  base0=LSB of Input  dbl_ovrd=off  block_type=slice
  slice_ts_tvg_en : xbsIndex_r4/Slice  nbits=1  boolean_output=on  mode=Lower Bit Location + Width  bit1=0  base1=MSB of Input  bit0=10  base0=LSB of Input  dbl_ovrd=off  block_type=slice
  slice_tvg_adc0 : xbsIndex_r4/Slice  nbits=1  boolean_output=on  mode=Lower Bit Location + Width  bit1=0  base1=MSB of Input  bit0=23  base0=LSB of Input  dbl_ovrd=off  block_type=slice
  slice_tvg_adc1 : xbsIndex_r4/Slice  nbits=1  boolean_output=on  mode=Lower Bit Location + Width  bit1=0  base1=MSB of Input  bit0=22  base0=LSB of Input  dbl_ovrd=off  block_type=slice
  slice_unpack_debug_reset : xbsIndex_r4/Slice  nbits=1  boolean_output=on  mode=Lower Bit Location + Width  bit1=0  base1=MSB of Input  bit0=16  base0=LSB of Input  dbl_ovrd=off  block_type=slice
  in_sys_rst : Outport
  in_status_clr : Outport  Port=2
  in_gbe_rst : Outport  Port=3
  in_gbe_txen : Outport  Port=4
  in_tvg_adc0 : Outport  Port=5
  in_tvg_adc1 : Outport  Port=6
  in_cnt_rst : Outport  Port=7
  in_gbe_cnt_rst : Outport  Port=8
  in_adc_snap_arm : Outport  Port=9
  in_adc_snap_trig_select : Outport  Port=10
  in_ct_tvg_en : Outport  Port=11
  in_unpack_debug_reset : Outport  Port=12
  in_cd_bypass : Outport  Port=13
  in_gbe_stopmux : Outport  Port=14
  in_pfb_bypass : Outport  Port=15
  in_ts_tvg_en : Outport  Port=16
  in_force_gbe_txen : Outport  Port=17
  in_snap_stop_mux_sel : Outport  Port=18
  in_snap_reord_mux_we_sel : Outport  Port=19
  in_local_time_source : Outport  Port=20
  in_local_time_capture : Outport  Port=21
  in_time_diff_check_en : Outport  Port=22
  in_auto_rst_enable : Outport  Port=23
  in_pipeline_stall : Outport  Port=24
  wires:
  s_c_nbe_m32k_v9_control_user_data_out/1 -> io_delay/1
  sim_add/1 -> s_c_nbe_m32k_v9_control_user_data_out/1
  sim_1/1 -> convert1_1/1
  convert1_1/1 -> convert2_1/1
  convert2_1/1 -> gain_1/1
  gain_1/1 -> sim_add/1
  io_delay/1 -> slice_sys_rst/1, slice_status_clr/1, slice_gbe_rst/1, slice_gbe_txen/1, slice_tvg_adc0/1, slice_tvg_adc1/1, slice_cnt_rst/1, slice_gbe_cnt_rst/1, slice_adc_snap_arm/1, slice_adc_snap_trig_select/1, slice_ct_tvg_en/1, slice_unpack_debug_reset/1, slice_cd_bypass/1, slice_gbe_stopmux/1, slice_pfb_bypass/1, slice_ts_tvg_en/1, slice_force_gbe_txen/1, slice_snap_stop_mux_sel/1, slice_snap_reord_mux_we_sel/1, slice_local_time_source/1, slice_local_time_capture/1, slice_time_diff_check_en/1, slice_auto_rst_enable/1, slice_pipeline_stall/1
  slice_sys_rst/1 -> in_sys_rst/1
  sim_2/1 -> convert1_2/1
  convert1_2/1 -> convert2_2/1
  convert2_2/1 -> gain_2/1
  gain_2/1 -> sim_add/2
  slice_status_clr/1 -> in_status_clr/1
  sim_3/1 -> convert1_3/1
  convert1_3/1 -> convert2_3/1
  convert2_3/1 -> gain_3/1
  gain_3/1 -> sim_add/3
  slice_gbe_rst/1 -> in_gbe_rst/1
  sim_4/1 -> convert1_4/1
  convert1_4/1 -> convert2_4/1
  convert2_4/1 -> gain_4/1
  gain_4/1 -> sim_add/4
  slice_gbe_txen/1 -> in_gbe_txen/1
  sim_5/1 -> convert1_5/1
  convert1_5/1 -> convert2_5/1
  convert2_5/1 -> gain_5/1
  gain_5/1 -> sim_add/5
  slice_tvg_adc0/1 -> in_tvg_adc0/1
  sim_6/1 -> convert1_6/1
  convert1_6/1 -> convert2_6/1
  convert2_6/1 -> gain_6/1
  gain_6/1 -> sim_add/6
  slice_tvg_adc1/1 -> in_tvg_adc1/1
  sim_7/1 -> convert1_7/1
  convert1_7/1 -> convert2_7/1
  convert2_7/1 -> gain_7/1
  gain_7/1 -> sim_add/7
  slice_cnt_rst/1 -> in_cnt_rst/1
  sim_8/1 -> convert1_8/1
  convert1_8/1 -> convert2_8/1
  convert2_8/1 -> gain_8/1
  gain_8/1 -> sim_add/8
  slice_gbe_cnt_rst/1 -> in_gbe_cnt_rst/1
  sim_9/1 -> convert1_9/1
  convert1_9/1 -> convert2_9/1
  convert2_9/1 -> gain_9/1
  gain_9/1 -> sim_add/9
  slice_adc_snap_arm/1 -> in_adc_snap_arm/1
  sim_10/1 -> convert1_10/1
  convert1_10/1 -> convert2_10/1
  convert2_10/1 -> gain_10/1
  gain_10/1 -> sim_add/10
  slice_adc_snap_trig_select/1 -> reint10/1
  reint10/1 -> in_adc_snap_trig_select/1
  sim_11/1 -> convert1_11/1
  convert1_11/1 -> convert2_11/1
  convert2_11/1 -> gain_11/1
  gain_11/1 -> sim_add/11
  slice_ct_tvg_en/1 -> reint11/1
  reint11/1 -> in_ct_tvg_en/1
  sim_12/1 -> convert1_12/1
  convert1_12/1 -> convert2_12/1
  convert2_12/1 -> gain_12/1
  gain_12/1 -> sim_add/12
  slice_unpack_debug_reset/1 -> in_unpack_debug_reset/1
  sim_13/1 -> convert1_13/1
  convert1_13/1 -> convert2_13/1
  convert2_13/1 -> gain_13/1
  gain_13/1 -> sim_add/13
  slice_cd_bypass/1 -> reint13/1
  reint13/1 -> in_cd_bypass/1
  sim_14/1 -> convert1_14/1
  convert1_14/1 -> convert2_14/1
  convert2_14/1 -> gain_14/1
  gain_14/1 -> sim_add/14
  slice_gbe_stopmux/1 -> reint14/1
  reint14/1 -> in_gbe_stopmux/1
  sim_15/1 -> convert1_15/1
  convert1_15/1 -> convert2_15/1
  convert2_15/1 -> gain_15/1
  gain_15/1 -> sim_add/15
  slice_pfb_bypass/1 -> reint15/1
  reint15/1 -> in_pfb_bypass/1
  sim_16/1 -> convert1_16/1
  convert1_16/1 -> convert2_16/1
  convert2_16/1 -> gain_16/1
  gain_16/1 -> sim_add/16
  slice_ts_tvg_en/1 -> in_ts_tvg_en/1
  sim_17/1 -> convert1_17/1
  convert1_17/1 -> convert2_17/1
  convert2_17/1 -> gain_17/1
  gain_17/1 -> sim_add/17
  slice_force_gbe_txen/1 -> in_force_gbe_txen/1
  sim_18/1 -> convert1_18/1
  convert1_18/1 -> convert2_18/1
  convert2_18/1 -> gain_18/1
  gain_18/1 -> sim_add/18
  slice_snap_stop_mux_sel/1 -> reint18/1
  reint18/1 -> in_snap_stop_mux_sel/1
  sim_19/1 -> convert1_19/1
  convert1_19/1 -> convert2_19/1
  convert2_19/1 -> gain_19/1
  gain_19/1 -> sim_add/19
  slice_snap_reord_mux_we_sel/1 -> reint19/1
  reint19/1 -> in_snap_reord_mux_we_sel/1
  sim_20/1 -> convert1_20/1
  convert1_20/1 -> convert2_20/1
  convert2_20/1 -> gain_20/1
  gain_20/1 -> sim_add/20
  slice_local_time_source/1 -> reint20/1
  reint20/1 -> in_local_time_source/1
  sim_21/1 -> convert1_21/1
  convert1_21/1 -> convert2_21/1
  convert2_21/1 -> gain_21/1
  gain_21/1 -> sim_add/21
  slice_local_time_capture/1 -> in_local_time_capture/1
  sim_22/1 -> convert1_22/1
  convert1_22/1 -> convert2_22/1
  convert2_22/1 -> gain_22/1
  gain_22/1 -> sim_add/22
  slice_time_diff_check_en/1 -> in_time_diff_check_en/1
  sim_23/1 -> convert1_23/1
  convert1_23/1 -> convert2_23/1
  convert2_23/1 -> gain_23/1
  gain_23/1 -> sim_add/23
  slice_auto_rst_enable/1 -> in_auto_rst_enable/1
  sim_24/1 -> convert1_24/1
  convert1_24/1 -> convert2_24/1
  convert2_24/1 -> gain_24/1
  gain_24/1 -> sim_add/24
  slice_pipeline_stall/1 -> in_pipeline_stall/1
